simulink model "DCFastCharger"  (R2026b)
settings: Solver=ode23t  StopTime=simulation.simTime  MaxStep=1/(5*inverter.SwitchFrequency)  AbsTol=1e-3
PreLoadFcn:
  | run('DCFastChargerData.mlx');
undefined symbols (not defined in the file or in its folder): battery, inverter, rectifier
libraries: nesl_utility x34, fl_lib x22, ee_lib x14, eePwmGenerator x2, eeTransforms x2, batteryecm_lib x1, eeSinusoidalMeasurement x1, slpidlib x1, eePwmGeneratorThreeLevel x1, eePwmGeneratorTwoLevel x1, simulink_extras x1
(part 2 of 3)

== system DCFastCharger/EV Battery/EV Battery ==
  Battery (Table-Based) : batteryecm_lib/Battery (Table-Based)  PartSpecification="{\"CollectionId\":\"MW.SimscapeBatteryShared\",\"CollectionVersion\":\"1.0.0\",\"DatasetId\":\"Panasonic|NCR18650PF|simscape.battery.batteryTableBased\",\"DisplayName\":\"Panasonic:NCR18650PF\"}"  SOC_vec=[0 0.01 0.02 0.03 0.04 0.05 0.06 0.07 0.08 0.09 0.1 0.11 0.12 0.13 0.14 0.15 0.16 0.17 0.18 0.19 0.2 0.21 0.22 0.23 0.24 0.25 0.26 0.27 0.28 0.29 0.3 0.31 0.32 0.33 0.34 0.35 0.36 0.37 0.38 0.39 0.4 0.41 0.42 0.43 0.44 0.45 0.46 0.47 0.48 0.49 0.5 0.51 0.52 0.53 0.54 0.55 0.56 0.57 0.58 0.59 0.6 0.61 0.62 0.63 0.64 0.65 0.66 0.67 0.68 0.69 0.7 0.71 0.72 0.73 0.74 0.75 0.76 0.77 0.78 0.79 0.8 0.81 0.82 0.83 0.84 0.85 0.86 0.87 0.88 0.89 0.9 0.91 0.92 0.93 0.94 0.95 0.96 0.97 0.98 0.99 1]  T_dependence=simscape.enum.tablebattery.temperature_dependence.no  prm_dir=simscape.enum.tablebattery.prm_dir.noCurrentDirectionality  T_vec=[-10 0 25 45] degC  V0_mat=[2.9250925086225 2.9250925086225 2.9250925086225 2.9250925086225;3.02630036129653 3.02630036129653 3.02630036129653 3.02630036129653;3.10541208785785 3.10541208785785 3.10541208785785 3.10541208785785;3.16593241088406 3.16593241088406 3.16593241088406 3.16593241088406;3.21032916159511 3.21032916159511 3.21032916159511 3.21032916159511;3.25202417776279 3.25202417776279 3.25202417776279 3.25202417776279;3.27764615366987 3.27764615366987 3.27764615366987 3.27764615366987;3.30010470561178 3.30010470561178 3.30010470561178 3.30010470561178;3.32101021333279 3.32101021333279 3.32101021333279 3.32101021333279;3.33984622770258 3.33984622770258 3.33984622770258 3.33984622770258;3.35585830950675 3.35585830950675 3.35585830950675 3.35585830950675;3.37108925119603 3.37108925119603 3.37108925119603 3.37108925119603;3.3859421763038 3.3859421763038 3.3859421763038 3.3859421763038;3.39949357655528 3.39949357655528 3.39949357655528 3.39949357655528;3.41188533180246 3.41188533180246 3.41188533180246 3.41188533180246;3.42508750933082 3.42508750933082 3.42508750933082 3.42508750933082;3.43732483114827 3.43732483114827 3.43732483114827 3.43732483114827;3.44838610292672 3.44838610292672 3.44838610292672 3.44838610292672;3.45940404792364 3.45940404792364 3.45940404792364 3.45940404792364;3.46945718604369 3.46945718604369 3.46945718604369 3.46945718604369;3.4756511424782 3.4756511424782 3.4756511424782 3.4756511424782;3.48092723774567 3.48092723774567 3.48092723774567 3.48092723774567;3.48828844475697 3.48828844475697 3.48828844475697 3.48828844475697;3.49727445600775 3.49727445600775 3.49727445600775 3.49727445600775;3.50602219248741 3.50602219248741 3.50602219248741 3.50602219248741;3.51277142257531 3.51277142257531 3.51277142257531 3.51277142257531;3.5189897231308 3.5189897231308 3.5189897231308 3.5189897231308;3.52519494567954 3.52519494567954 3.52519494567954 3.52519494567954;3.53104467138329 3.53104467138329 3.53104467138329 3.53104467138329;3.53631377637871 3.53631377637871 3.53631377637871 3.53631377637871;3.54093819602626 3.54093819602626 3.54093819602626 3.54093819602626;3.54463024006975 3.54463024006975 3.54463024006975 3.54463024006975;3.54855792050501 3.54855792050501 3.54855792050501 3.54855792050501;3.55281403232742 3.55281403232742 3.55281403232742 3.55281403232742;3.55817391786706 3.55817391786706 3.55817391786706 3.55817391786706;3.56415253483575 3.56415253483575 3.56415253483575 3.56415253483575;3.56997687090312 3.56997687090312 3.56997687090312 3.56997687090312;3.57540644773372 3.57540644773372 3.57540644773372 3.57540644773372;3.58072477562415 3.58072477562415 3.58072477562415 3.58072477562415;3.58617648767287 3.58617648767287 3.58617648767287 3.58617648767287;3.59255537492352 3.59255537492352 3.59255537492352 3.59255537492352;3.59925786836004 3.59925786836004 3.59925786836004 3.59925786836004;3.6059599902444 3.6059599902444 3.6059599902444 3.6059599902444;3.61253369195548 3.61253369195548 3.61253369195548 3.61253369195548;3.61908508495676 3.61908508495676 3.61908508495676 3.61908508495676;3.62459685737123 3.62459685737123 3.62459685737123 3.62459685737123;3.62997084407271 3.62997084407271 3.62997084407271 3.62997084407271;3.63600645659379 3.63600645659379 3.63600645659379 3.63600645659379;3.64260961230588 3.64260961230588 3.64260961230588 3.64260961230588;3.64905571343015 3.64905571343015 3.64905571343015 3.64905571343015;3.65538413005486 3.65538413005486 3.65538413005486 3.65538413005486;3.66209665206491 3.66209665206491 3.66209665206491 3.66209665206491;3.66960310665593 3.66960310665593 3.66960310665593 3.66960310665593;3.67782215533979 3.67782215533979 3.67782215533979 3.67782215533979;3.68577251249088 3.68577251249088 3.68577251249088 3.68577251249088;3.69607105582974 3.69607105582974 3.69607105582974 3.69607105582974;3.70665559836365 3.70665559836365 3.70665559836365 3.70665559836365;3.71697762414446 3.71697762414446 3.71697762414446 3.71697762414446;3.72601099321076 3.72601099321076 3.72601099321076 3.72601099321076 ...(+2844 chars)] V  V0_vec=[2.9250925086225 3.02630036129653 3.10541208785785 3.16593241088406 3.21032916159511 3.25202417776279 3.27764615366987 3.30010470561178 3.32101021333279 3.33984622770258 3.35585830950675 3.37108925119603 3.3859421763038 3.39949357655528 3.41188533180246 3.42508750933082 3.43732483114827 3.44838610292672 3.45940404792364 3.46945718604369 3.4756511424782 3.48092723774567 3.48828844475697 3.49727445600775 3.50602219248741 3.51277142257531 3.5189897231308 3.52519494567954 3.53104467138329 3.53631377637871 3.54093819602626 3.54463024006975 3.54855792050501 3.55281403232742 3.55817391786706 3.56415253483575 3.56997687090312 3.57540644773372 3.58072477562415 3.58617648767287 3.59255537492352 3.59925786836004 3.6059599902444 3.61253369195548 3.61908508495676 3.62459685737123 3.62997084407271 3.63600645659379 3.64260961230588 3.64905571343015 3.65538413005486 3.66209665206491 3.66960310665593 3.67782215533979 3.68577251249088 3.69607105582974 3.70665559836365 3.71697762414446 3.72601099321076 3.73441114732962 3.74311002352401 3.75294627542582 3.76247271262466 3.77151242602685 3.78040087631196 3.79005401630221 3.79990949046456 3.80976496462691 3.81844612732862 3.82578802176443 3.83313829687425 3.84080281949238 3.84973459076441 3.85949329030869 3.86965559240319 3.87924489617679 3.88819434423151 3.89590288247261 3.90359081518304 3.91379255081804 3.92466354434184 3.9366161325385 3.95005027786179 3.96305146054116 3.97214053014382 3.98120257186703 3.99267995044399 4.0057555337863 4.0188391070389 4.03188069898376 4.04441045486762 4.05587613526738 4.06606826108443 4.07458148513164 4.08216556084643 4.08994198301214 4.10139357870482 4.11503704946696 4.13270033629767 4.15282395048316 4.17387289866414] V  V_range=[0, inf] V  R0_mat=[0.158948722548683 0.155965220476233 0.0642584048974491 0.156271637839508;0.164094056100913 0.155561872039019 0.0643716270460056 0.0958858667534425;0.16590247791362 0.150196791550074 0.063971690534484 0.0735783105788718;0.164336402457897 0.145157421371546 0.0634227939708557 0.0603478425562904;0.162194103534027 0.137561513429308 0.0626187357617236 0.0554701940184629;0.161368428396527 0.132847642820159 0.0622925177341011 0.0565695495484196;0.154034534555668 0.126124135972156 0.0608902569786277 0.0547834384667639;0.150348957772332 0.11992991718736 0.0592086978048456 0.0546076326919676;0.146678161591533 0.114221598629678 0.0583937154824633 0.0553174331388643;0.143764862122133 0.1117675900648 0.057496531429448 0.0567839252512895;0.141557404155717 0.108267680549691 0.0573966942403751 0.0568973079738719;0.139111638730854 0.10588448132351 0.0571494121217046 0.0563386051707534;0.137029789271551 0.10371863599948 0.0568904518955565 0.0568492069290691;0.134465893569179 0.102157603100912 0.0566162508651665 0.0573623269867748;0.133579806251124 0.101182159975048 0.0563201629222844 0.0575820103565126;0.133163032374253 0.100506873249622 0.0564506791916006 0.0591218449352567;0.132701252660884 0.099863696339387 0.0563243957272469 0.0603043255469938;0.131974699165714 0.0988544564628729 0.0561368224553059 0.0604335920006752;0.131283115762638 0.098955481127068 0.0562749855286881 0.0603849408722603;0.130548646804137 0.099375021703539 0.0562019955818807 0.0601584729212836;0.128384851295437 0.0983652357298114 0.0555274629478928 0.0592378223566733;0.126118815339946 0.0970669163577878 0.0546888535605859 0.0579772232116761;0.125402797723443 0.0966018361754667 0.054265365781618 0.057400894490884;0.125288559454898 0.096738535341105 0.0540037545839983 0.0569904797117699;0.125047401593192 0.0967965349271084 0.0536899957091979 0.0564918150174259;0.124051599285487 0.0961581839164014 0.0533086284567699 0.0554970632508009;0.12285915641022 0.0953231923381314 0.0530642654231626 0.054870770374079;0.122165505140544 0.094483357053662 0.0528170401995282 0.0542396337911578;0.121494072509647 0.0935118562710458 0.0525235778530978 0.053212217478928;0.120601470615727 0.0925622611521829 0.0520471214590463 0.0519633792021407;0.119286253401761 0.091460027942767 0.0514017212712578 0.0507774032613698;0.117625711889992 0.0900124704355474 0.0505504728406427 0.0494999445481573;0.116099177219541 0.088652185666025 0.049830956429225 0.0490253291641116;0.114900842886945 0.0876321360266284 0.0493618778947113 0.0489723769096966;0.114111313634808 0.0873497188498393 0.0490976398787349 0.0493282297357397;0.113550944171205 0.0872964614615855 0.048915118220372 0.0492640332618821;0.112988973186793 0.0871860629987678 0.048614953173201 0.0489039680872592;0.112297629639516 0.0869949880800038 0.0482896295727264 0.048407984264869;0.111565082781067 0.0870678281013333 0.0479473144926267 0.048233027492356;0.110761242109476 0.0871900696627706 0.0477067084656926 0.0481074722599508;0.110212729124657 0.0876557094471428 0.0476555994749632 0.0483253152504805;0.109784070282755 0.0873084934166727 0.0476617367023012 0.0482979562377831;0.109503678016475 0.0860654941887924 0.0476677926135098 0.0477344062008158;0.109268014836562 0.0847749319337712 0.0476696468980676 0.0471232931367077;0.109024089171536 0.0838029485664093 0.0476752475967437 0.0465039175874869;0.108621493141403 0.0835326079948486 0.0474506512594163 0.0461687494231811;0.108259397918414 0.0832112356777327 0.0471837257520344 0.0458650723508987;0.108008944918365 0.0831349099604705 0.0468394367793266 0.0455774893634449;0.107209504544399 0.082814101209584 0.0466240014760817 0.0450730540518787;0.106351895804571 0.0823498486862532 0.0464022435243735 0.0445104503744493;0.105450700213058 0.0818420093112374 0.0461547297057605 0.043898896196232;0.104474728336867 0.0815181360390074 0.045579722159839 0.0433287006666967;0.103783729089634 0.0816852711857715 0.0450589645831341 0.0430525542412283;0.103537470985121 0.0821163300706208 0.044701216779163 ...(+3502 chars)] Ohm  R0_vec=[0.0642584048974491 0.0643716270460056 0.063971690534484 0.0634227939708557 0.0626187357617236 0.0622925177341011 0.0608902569786277 0.0592086978048456 0.0583937154824633 0.057496531429448 0.0573966942403751 0.0571494121217046 0.0568904518955565 0.0566162508651665 0.0563201629222844 0.0564506791916006 0.0563243957272469 0.0561368224553059 0.0562749855286881 0.0562019955818807 0.0555274629478928 0.0546888535605859 0.054265365781618 0.0540037545839983 0.0536899957091979 0.0533086284567699 0.0530642654231626 0.0528170401995282 0.0525235778530978 0.0520471214590463 0.0514017212712578 0.0505504728406427 0.049830956429225 0.0493618778947113 0.0490976398787349 0.048915118220372 0.048614953173201 0.0482896295727264 0.0479473144926267 0.0477067084656926 0.0476555994749632 0.0476617367023012 0.0476677926135098 0.0476696468980676 0.0476752475967437 0.0474506512594163 0.0471837257520344 0.0468394367793266 0.0466240014760817 0.0464022435243735 0.0461547297057605 0.045579722159839 0.0450589645831341 0.044701216779163 0.0443326520857887 0.0445314146147127 0.045015739502721 0.0454894960834381 0.0456812234168713 0.0456928203147297 0.0455424443466032 0.0455233887186122 0.0454918606790689 0.0454039925420258 0.0452830196823913 0.0453842814819192 0.0455361622547251 0.0456880430275314 0.0456524416563551 0.0454382214701634 0.0452225970388179 0.0450757473146783 0.0448448857727635 0.0447127937510717 0.0447342410972344 0.0448403278985325 0.0450878835664416 0.0450853981911946 0.0450820832857262 0.0456224791026564 0.0458434697709894 0.046286077419994 0.0470885819136486 0.0477828468023542 0.0475520781260466 0.0472569254085986 0.0474663234338054 0.0479591925321213 0.0484565832495922 0.0490028384423885 0.0495284883187202 0.0497251543915884 0.0496855026515378 0.0492826811538264 0.0486578614415746 0.0474486947337877 0.0465126146130306 0.0457818101518658 0.0456572937139443 0.0412205205929347 0.0351051518441569] Ohm  R0_dis_mat=[0.03 0.015 0.002;0.04 0.017 0.008;0.039 0.012 0.006;0.027 0.013 0.021] % Parameter not set Ohm  R0_dis_vec=[0.015 0.017 0.012 0.013] % Parameter not set Ohm  R0_ch_mat=[0.03 0.015 0.002;0.04 0.017 0.008;0.039 0.012 0.006;0.027 0.013 0.021] % Parameter not set Ohm  R0_ch_vec=[0.015 0.017 0.012 0.013] % Parameter not set Ohm  AH=2.73516665928367 hr*A  prm_leak=simscape.enum.tablebattery.prm_leak.disabled  Rleak_vec=[8000 7000 6000] % Parameter not set Ohm  Rleak=7000 % Parameter not set Ohm  extrapolation_option=simscape.enum.extrapolation.nearest  SOC_port=simscape.enum.tablebattery.enable.yes  prm_dyn=simscape.enum.tablebattery.prm_dyn.off  R1_mat=[0.089 0.076 0.01;0.042 0.022 0.099;0.019 0.007 0.002;0.051 0.043 0.029] % Parameter not set Ohm  R1_vec=[0.076 0.022 0.007 0.043] % Parameter not set Ohm  tau1_mat=[44 148 235;93 110 1000;19 27 133;0.5 22 3] % Parameter not set s  tau1_vec=[148 110 27 22] % Parameter not set s  R2_mat=[0.014 0.382 0.407;0.028 0.006 0.007;0.014 0.007 0.006;0.333 0.956 0.912] % Parameter not set Ohm  R2_vec=[0.382 0.006 0.007 0.956] % Parameter not set Ohm  tau2_mat=[1 44 5644;11 24 506;2 14 330;3310 13419 30216] % Parameter not set s  tau2_vec=[44 24 14 13419] % Parameter not set s  R3_mat=[0.014 0.382 0.407;0.028 0.006 0.007;0.014 0.007 0.006;0.333 0.956 0.912] % Parameter not set Ohm  R3_vec=[0.382 0.006 0.007 0.956] % Parameter not set Ohm  tau3_mat=[1 44 5644;11 24 506;2 14 330;3310 13419 30216] % Parameter not set s  tau3_vec=[44 24 14 13419] % Parameter not set s  R4_mat=[0.014 0.382 0.407;0.028 0.006 0.007;0.014 0.007 0.006;0.333 0.956 0.912] % Parameter not set Ohm  R4_vec=[0.382 0.006 0.007 0.956] % Parameter not set Ohm  tau4_mat=[1 44 5644;11 24 506;2 14 330;3310 13419 30216] % Parameter not set s  tau4_vec=[44 24 14 13419] % Parameter not set s  R5_mat=[0.014 0.382 0.407;0.028 0.006 0.007;0.014 0.007 0.006;0.333 0.956 0.912] % Parameter not set Ohm  R5_vec=[0.382 0.006 0.007 0.956] % Parameter not set Ohm  tau5_mat=[1 44 5644;11 24 506;2 14 330;3310 13419 30216] % Parameter not set s  tau5_vec=[44 24 14 13419] % Parameter not set s  prm_fade=simscape.enum.tablebattery.prm_fade.tableN  N0=100 % Parameter not set  dV0=0 % Parameter not set  dR0=0 % Parameter not set  dAH=0 % Parameter not set  dRleak=0 % Parameter not set  dR1=0 % Parameter not set  dR2=0 % Parameter not set  dR3=0 % Parameter not set  dR4=0 % Parameter not set  dR5=0 % Parameter not set  N0vec=[1 7 13 19 25 31 37 43 49 55 61 67 73 79 85 91 97 103 109 115 121 127 133 139 145 151 157 163 169 175 181 187 193 199 205 211 217 223 229 235 241 247 253 259 265 271 277 283 289 295 301 307 313 319 325 331 337 343 349 355 361 367 373 379 385 391 397 403 409 415 421 427 433 439 445 451 457 463 469 475 481 487 493 499]  Tfadevec=[298.15 323.15] % Parameter not set K  dV0vec=[0 -0.205322446679001 -0.410644893358002 -0.611058438675835 -0.807354693721955 -1.0015461710045 -1.17384310657063 -1.34614004213677 -1.47740012287432 -1.58387836723114 -1.690356611588 -1.78714189934731 -1.87651401189101 -1.96588612443468 -2.04101080690197 -2.10170062652461 -2.16239044614726 -2.21633350400211 -2.26428234838279 -2.31223119276347 -2.36018003714415 -2.41171229286392 -2.46553549695213 -2.51935870104035 -2.57318190512856 -2.64508715419502 -2.72179418719877 -2.79850122020252 -2.88122798263413 -2.96751992414094 -3.05381186564772 -3.14366470722484 -3.23796499505138 -3.33226528287793 -3.38092510003549 -3.4273752475407 -3.47468340383756 -3.52199156013442 -3.56929971643126 -3.61660787272814 -3.663916029025 -3.71122418532186 -3.76958571632676 -3.83114472817411 -3.89270374002147 -3.95426275186883 -4.01582176371619 -4.07735052835229 -4.13887194718341 -4.20039336601454 -4.26007865261728 -4.31160679119979 -4.36044442770985 -4.40567437565134 -4.45090432359283 -4.49613427153431 -4.54136421947579 -4.58659416741728 -4.62903918136233 -4.6691583474524 -4.70927751354245 -4.74939667963251 -4.78951584572256 -4.82963501181263 -4.86986314897544 -4.91010197198366 -4.95034079499188 -4.98044487353192 -4.99960776219833 -5.01877065086475 -5.03793353953117 -5.05972954523592 -5.08714051545705 -5.11455148567819 -5.14196245589932 -5.17147950123752 -5.20235900192375 -5.23323850260996 -5.26411800329619 -5.29499750398241 -5.32587700466864 -5.35675650535486 -5.38847412791779 -5.42038197122406]  dR0vec=[0;0;0;0;0;0;0;0;0;0;0;0;0;0;0;0;0;0;0;0;0;0;0;0;0;0;0;0;0;0;0;0;0;0;0;0;0;0;0;0;0;0;0;0;0;0;0;0;0;0;0;0;0;0;0;0;0;0;0;0;0;0;0;0;0;0;0;0;0;0;0;0;0;0;0;0;0;0;0;0;0;0;0;0] % Parameter not set  dAHvec=[0 -0.407141386976734 -0.814282773953468 -1.22142416093019 -1.62856554790692 -2.03570693488365 -2.44284832186039 -2.84998970883712 -3.20734856882233 -3.53309167786423 -3.85883478690612 -4.18457789594802 -4.51032100498989 -4.8360641140318 -5.1618072230737 -5.48755033211559 -5.81329344115748 -6.10543218183984 -6.36931718194932 -6.63320218205879 -6.89708718216827 -7.16097218227776 -7.42485718238722 -7.6887421824967 -7.95262718260619 -8.25489660762765 -8.56902676255148 -8.8831569174753 -9.19728707239912 -9.51141722732295 -9.82554738224679 -10.1396775371706 -10.4538076920944 -10.7679378470183 -10.9300319005421 -11.0814384407007 -11.2328449808593 -11.3842515210179 -11.5356580611765 -11.6870646013351 -11.8384711414938 -11.9898776816524 -12.176092947695 -12.3724762187309 -12.5688594897668 -12.7652427608027 -12.9616260318386 -13.1580093028745 -13.3543925739104 -13.5507758449463 -13.7412979759122 -13.9057815752421 -14.0702651745719 -14.2347487739018 -14.3992323732316 -14.5637159725615 -14.7281995718913 -14.8926831712212 -15.0595765368119 -15.2443608328623 -15.4291451289128 -15.6139294249632 -15.7987137210137 -15.9834980170641 -16.1682823131146 -16.353066609165 -16.5378509052155 -16.6760945352573 -16.7640941492568 -16.8520937632563 -16.9400933772558 -17.0280929912553 -17.1160926052547 -17.2040922192542 -17.2920918332537 -17.3868527474137 -17.4859876601498 -17.585122572886 -17.6842574856221 -17.7833923983582 -17.8825273110943 -17.9816622238304 -18.0807971365665 -18.1799320493027]  dRleakvec=[0 0 0] % Parameter not set  dR1vec=[0 0 0] % Parameter not set  dR2vec=[0 0 0] % Parameter not set  dR3vec=[0 0 0] % Parameter not set  dR4vec=[0 0 0] % Parameter not set  dR5vec=[0 0 0] % Parameter not set  dV0mat=[0 0;0 0;0 0] % Parameter not set  dR0mat=[0 0;0 0;0 0] % Parameter not set  dAHmat=[0 0;0 0;0 0] % Parameter not set  dRleakmat=[0 0;0 0;0 0] % Parameter not set  dR1mat=[0 0;0 0;0 0] % Parameter not set  dR2mat=[0 0;0 0;0 0] % Parameter not set  dR3mat=[0 0;0 0;0 0] % Parameter not set  dR4mat=[0 0;0 0;0 0] % Parameter not set  dR5mat=[0 0;0 0;0 0] % Parameter not set  prm_age_modeling=simscape.enum.tablebattery.prm_age_modeling.equation  storage_dt_age_vec=0 % Parameter not set d  storage_T_age_vec=273 % Parameter not set K  prm_age_OCV=simscape.enum.tablebattery.prm_age_OCV.SOC  OCV_age=0.9 % Parameter not set  SOC_age=0.6 % Parameter not set  prm_age_resistance=simscape.enum.tablebattery.prm_age.disabled  OCV_scaling_age_resistance=2213400  OCV_offset_age_resistance=1632000  temp_exp_age_resistance=0.515833569 V  t_exp_age_resistance=0.75  T_age_vec_resistance=[273.15 298.15 323.15] K  dt_age_vec_resistance=[90 180 270 360] d  dR0_age_vec=[0 0 0] % Parameter not set  t_meas_dR0_age=100 % Parameter not set d  dR0_age_mat=[0 0 0;0 0 0;0 0 0;0 0 0] % Parameter not set  prm_age_capacity=simscape.enum.tablebattery.prm_age.disabled  OCV_scaling_age_capacity=1.5097e07  OCV_offset_age_capacity=8.3625e06  temp_exp_age_capacity=0.6011 V  t_exp_age_capacity=0.75  T_age_vec_capacity=[273.15, 298.15, 323.15] K  dt_age_vec_capacity=[90, 180, 270, 360] d  dAH_age_vec=[0, 0, 0]  t_meas_dAH_age=100 d  dAH_age_mat=[0, 0, 0; 0, 0, 0; 0, 0, 0; 0, 0, 0]  thermal_port=simscape.enum.thermaleffects.omit  temperature=298.15 K  thermal_mass=30000 J/K  i_specify=off  i_priority=None  i=0 A  i_nominal_specify=off  i_nominal_value=1  i_nominal_unit=A  v_specify=off  v_priority=None  v=0 V  v_nominal_specify=off  v_nominal_value=1  v_nominal_unit=V  stateOfCharge_specify=on  stateOfCharge_priority=High  stateOfCharge=battery.initialSOC  stateOfCharge_nominal_specify=off  stateOfCharge_nominal_value=1  stateOfCharge_nominal_unit=1  num_cycles_specify=off  num_cycles_priority=High  num_cycles=0  num_cycles_nominal_specify=off  num_cycles_nominal_value=1  num_cycles_nominal_unit=1  cell_temperature_specify=off  cell_temperature_priority=High  cell_temperature=298.15 K  cell_temperature_nominal_specify=off  cell_temperature_nominal_value=1  cell_temperature_nominal_unit=K
      settings: AttributesFormatString=Panasonic:NCR18650PF
  "Number of cells in series " : fl_lib/Electrical/Electrical Sources/Voltage-Controlled Voltage Source  K=-1*battery.cellsInSeries  v1_specify=off  v1_priority=None  v1=0 V  v1_nominal_specify=off  v1_nominal_value=1  v1_nominal_unit=V  v2_specify=off  v2_priority=None  v2=0 V  v2_nominal_specify=off  v2_nominal_value=1  v2_nominal_unit=V
  Number of strings in parallel : fl_lib/Electrical/Electrical Sources/Current-Controlled Current Source  K=-1*(battery.batteryStringsInParallel-1)  i1_specify=off  i1_priority=None  i1=0 A  i1_nominal_specify=off  i1_nominal_value=1  i1_nominal_unit=A  i2_specify=off  i2_priority=None  i2=0 A  i2_nominal_specify=off  i2_nominal_value=1  i2_nominal_unit=A
  PS-Simulink Converter : nesl_utility/PS-Simulink Converter  PhysicalDomain=network_engine_domain  SubClassName=ps_output  LeftPortType=input  RightPortType=output  PseudoPeriodic=off  Frequencies=[]  VectorFormat=1-D array  Unit=inherit  AffineConversion=off
  + : PMIOPort  Side=Left
  - : PMIOPort  Port=2  Side=Right
  SOC : Outport
  wires:
  PS-Simulink Converter/1 -> SOC/1
  connections:
  "Number of cells in series "/RConn2 -- "Number of cells in series "/RConn1 -- Battery (Table-Based)/LConn1
  "Number of cells in series "/LConn1 -- Number of strings in parallel/LConn2 -- -/RConn1 -- Battery (Table-Based)/RConn1
  Number of strings in parallel/RConn1 -- Number of strings in parallel/RConn2 -- +/RConn1
  Number of strings in parallel/LConn1 -- "Number of cells in series "/LConn2
  PS-Simulink Converter/LConn1 -- Battery (Table-Based)/LConn2

== system DCFastCharger/EV Battery/i ==
  Current Sensor : fl_lib/Electrical/Electrical Sensors/Current Sensor
  PS-Simulink Converter1 : nesl_utility/PS-Simulink Converter  PhysicalDomain=network_engine_domain  SubClassName=ps_output  LeftPortType=input  RightPortType=output  PseudoPeriodic=off  Frequencies=[]  VectorFormat=1-D array  Unit=1  AffineConversion=off
  Rate Transition : RateTransition  OutPortSampleTime=1/(10*inverter.SwitchFrequency)
  + : PMIOPort  Side=Left
  - : PMIOPort  Port=2  Side=Right
  I : Outport
  wires:
  Rate Transition/1 -> I/1
  PS-Simulink Converter1/1 -> Rate Transition/1
  connections:
  Current Sensor/RConn1 -- PS-Simulink Converter1/LConn1
  Current Sensor/RConn2 -- -/RConn1
  Current Sensor/LConn1 -- +/RConn1

== system DCFastCharger/EV Battery/v ==
  PS-Simulink Converter : nesl_utility/PS-Simulink Converter  PhysicalDomain=network_engine_domain  SubClassName=ps_output  LeftPortType=input  RightPortType=output  PseudoPeriodic=off  Frequencies=[]  VectorFormat=1-D array  Unit=1  AffineConversion=off
  Rate Transition : RateTransition  OutPortSampleTime=1/(10*inverter.SwitchFrequency)
  Voltage Sensor : fl_lib/Electrical/Electrical Sensors/Voltage Sensor
  + : PMIOPort  Side=Right
  - : PMIOPort  Port=2  Side=Left
  V : Outport
  wires:
  PS-Simulink Converter/1 -> Rate Transition/1
  Rate Transition/1 -> V/1
  connections:
  +/RConn1 -- Voltage Sensor/LConn1
  -/RConn1 -- Voltage Sensor/RConn2
  Voltage Sensor/RConn1 -- PS-Simulink Converter/LConn1

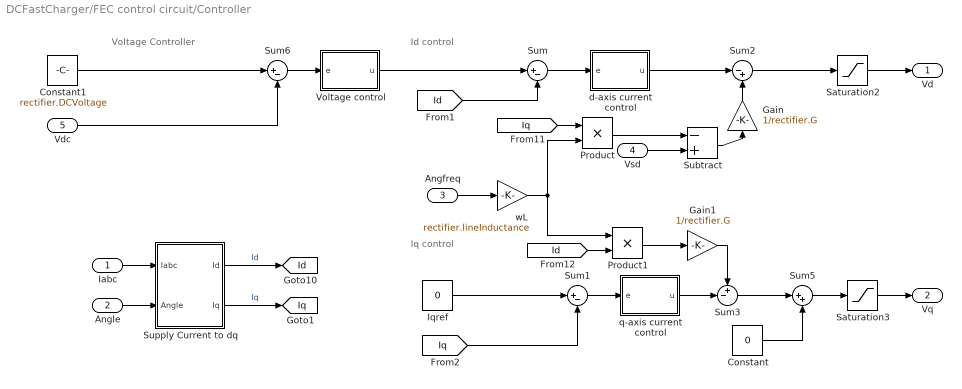
== system DCFastCharger/FEC control circuit/Controller ==
  note: Id control
  note: Voltage Controller
  note: Iq control
  Iabc : Inport
  Angle : Inport  Port=2
  Angfreq : Inport  Port=3
  Vsd : Inport  Port=4
  Vdc : Inport  Port=5
  Constant : Constant  Value=0
  Constant1 : Constant  Value=rectifier.DCVoltage
  Gain : Gain  Gain=1/rectifier.G
  Gain1 : Gain  Gain=1/rectifier.G
  Iqref : Constant  Value=0
  Product : Product
  Product1 : Product
  Saturation2 : Saturate  UpperLimit=4  LowerLimit=-3
  Saturation3 : Saturate  UpperLimit=1  LowerLimit=-1
  Subtract : Sum  Inputs=-+
  Sum : Sum  Inputs=|+-
  Sum1 : Sum  Inputs=|+-
  Sum2 : Sum  Inputs=|-+
  Sum3 : Sum  Inputs=+-|
  Sum5 : Sum  Inputs=|++
  Sum6 : Sum  Inputs=|+-
  Supply Current to dq : Subsystem
  Voltage control : Subsystem
  d-axis current control : Subsystem
  q-axis current control : Subsystem
  wL : Gain  Gain=rectifier.lineInductance
  Vd : Outport  VectorParamsAs1DForOutWhenUnconnected=off
  Vq : Outport  Port=2  VectorParamsAs1DForOutWhenUnconnected=off
  tag scope: Id=global, Iq=global
  wires:
  Sum1/1 -> q-axis current control/1(e)
  wL/1 -> Product/2, Product1/1
  [Id] -> Product1/2
  [Iq] -> Product/1
  Sum3/1 -> Sum5/1
  Sum2/1 -> Saturation2/1
  Sum5/1 -> Saturation3/1
  Angfreq/1 -> wL/1
  Constant/1 -> Sum5/2
  Vdc/1 -> Sum6/2
  Sum/1 -> d-axis current control/1(e)
  [Id] -> Sum/2
  d-axis current control/1(u) -> Sum2/1
  q-axis current control/1(u) -> Sum3/2
  Supply Current to dq/1(Id) -> [Id]  "Id"
  Supply Current to dq/2(Iq) -> [Iq]  "Iq"
  Sum6/1 -> Voltage control/1(e)
  Saturation3/1 -> Vq/1
  Saturation2/1 -> Vd/1
  Iqref/1 -> Sum1/1
  [Iq] -> Sum1/2
  Voltage control/1(u) -> Sum/1
  Constant1/1 -> Sum6/1
  Product1/1 -> Gain1/1
  Product/1 -> Subtract/1
  Vsd/1 -> Subtract/2
  Subtract/1 -> Gain/1
  Gain/1 -> Sum2/2
  Gain1/1 -> Sum3/1
  Iabc/1 -> Supply Current to dq/1(Iabc)
  Angle/1 -> Supply Current to dq/2(Angle)

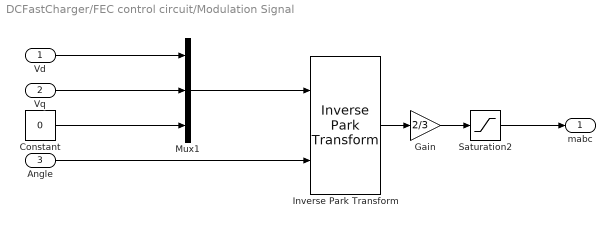
== system DCFastCharger/FEC control circuit/Modulation Signal ==
  Vd : Inport
  Vq : Inport  Port=2
  Angle : Inport  Port=3
  Constant : Constant  Value=0
  Gain : Gain  Gain=2/3
  Inverse Park Transform : eeTransforms/Inverse Park Transform  AxisAlignment=D-axis  PowerInvariant=off
  Mux1 : Mux  Inputs=3
  Saturation2 : Saturate  UpperLimit=1  LowerLimit=-1
  mabc : Outport  VectorParamsAs1DForOutWhenUnconnected=off
  wires:
  Gain/1 -> Saturation2/1
  Mux1/1 -> Inverse Park Transform/1
  Inverse Park Transform/1 -> Gain/1
  Constant/1 -> Mux1/3
  Vd/1 -> Mux1/1
  Vq/1 -> Mux1/2
  Angle/1 -> Inverse Park Transform/2
  Saturation2/1 -> mabc/1

== system DCFastCharger/Filter & AC measurements/PLL ==
  Vabc : Inport
  Constant : Constant  Value=pi/2
  Gain2 : Gain  Gain=2*pi
  "Sinusoidal measurement (PLL, Three-Phase)" : eeSinusoidalMeasurement/Sinusoidal Measurement (PLL, Three-Phase)  Kp_LF=0.05  Ki_LF=1  F0=rectifier.SystemFrequency  Theta0=0  Ts=rectifier.VoltageSensorT
  Subtract : Sum  Inputs=-+
  Vphm to Vsd : Gain  Gain=3/2
  w : Outport  VectorParamsAs1DForOutWhenUnconnected=off
  angle : Outport  Port=2  VectorParamsAs1DForOutWhenUnconnected=off
  Vsd : Outport  Port=3  VectorParamsAs1DForOutWhenUnconnected=off
  wires:
  "Sinusoidal measurement (PLL, Three-Phase)"/3 -> Vphm to Vsd/1
  Gain2/1 -> w/1
  "Sinusoidal measurement (PLL, Three-Phase)"/1 -> Gain2/1
  Vabc/1 -> "Sinusoidal measurement (PLL, Three-Phase)"/1
  Subtract/1 -> angle/1
  "Sinusoidal measurement (PLL, Three-Phase)"/2 -> Subtract/2
  Constant/1 -> Subtract/1
  Vphm to Vsd/1 -> Vsd/1

== system DCFastCharger/Front end converter/DC bus current sensor ==
  Current Sensor : fl_lib/Electrical/Electrical Sensors/Current Sensor
      settings: LogSimulationData=on
  PS-Simulink Converter1 : nesl_utility/PS-Simulink Converter  PhysicalDomain=network_engine_domain  SubClassName=ps_output  LeftPortType=input  RightPortType=output  PseudoPeriodic=off  Frequencies=[]  VectorFormat=1-D array  Unit=1  AffineConversion=off
  Sensor dynamics : TransferFcn  Numerator=1  Denominator=[1/(10*rectifier.SwitchFrequency) 1]
  + : PMIOPort  Side=Left
  - : PMIOPort  Port=2  Side=Right
  I : Outport
  wires:
  PS-Simulink Converter1/1 -> Sensor dynamics/1
  Sensor dynamics/1 -> I/1
  connections:
  Current Sensor/LConn1 -- +/RConn1
  PS-Simulink Converter1/LConn1 -- Current Sensor/RConn1
  Current Sensor/RConn2 -- -/RConn1

== system DCFastCharger/Front end converter/FEC ==
  m : Inport
  Vdc : Inport  Port=2
  Average : Subsystem  VariantControl=powerCircuit==0
  Three Level : Subsystem  VariantControl=powerCircuit==2
  Two Level : Subsystem  VariantControl=powerCircuit==1
  + : PMIOPort  Side=Right
  O : PMIOPort  Port=2  Side=Right
  - : PMIOPort  Port=3  Side=Right
  ABC : PMIOPort  Port=4  Side=Left

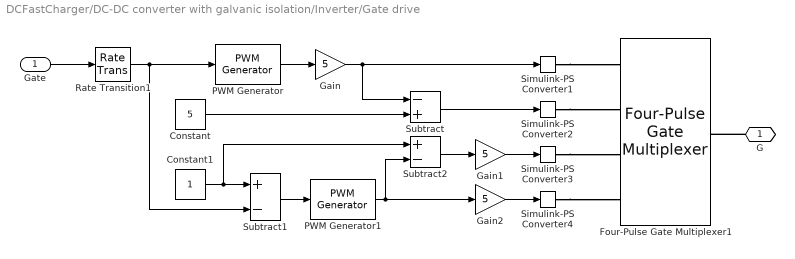
== system DCFastCharger/DC-DC converter with galvanic isolation/Inverter/Gate drive ==
  Gate : Inport
  Constant : Constant  Value=5
  Constant1 : Constant
  Four-Pulse Gate Multiplexer1 : ee_lib/Semiconductors & Converters/Converters/Four-Pulse Gate Multiplexer  port_option=ee.enum.controlport.ps
  Gain : Gain  Gain=5
  Gain1 : Gain  Gain=5
  Gain2 : Gain  Gain=5
  PWM Generator : eePwmGenerator/PWM Generator  CarrCount=Up  Tper=1/inverter.SwitchFrequency  Tdelay=0  Ts=1/(10*inverter.SwitchFrequency)
  PWM Generator1 : eePwmGenerator/PWM Generator  CarrCount=Up  Tper=1/inverter.SwitchFrequency  Tdelay=0  Ts=1/(10*inverter.SwitchFrequency)
  Rate Transition1 : RateTransition  OutPortSampleTime=1/(10*inverter.SwitchFrequency)
  Simulink-PS Converter{1..4} (4 alike) : nesl_utility/Simulink-PS Converter  PhysicalDomain=network_engine_domain  SubClassName=ps_input  LeftPortType=input  RightPortType=output  PseudoPeriodic=off  Frequencies=[]  NoiseDistribution=none  NoiseParameters=[]  Unit=1  AffineConversion=off  FilteringAndDerivatives=provide  SimscapeFilterOrder=1  InputFilterTimeConstant=0.001  UdotUserProvided=0
  Subtract : Sum  Inputs=-+
  Subtract1 : Sum  Inputs=+-
  Subtract2 : Sum  Inputs=+-
  G : PMIOPort  Side=Right
  wires:
  Rate Transition1/1 -> PWM Generator/1, Subtract1/2
  PWM Generator/1 -> Gain/1
  Constant/1 -> Subtract/2
  Gain/1 -> Simulink-PS Converter1/1, Subtract/1
  Subtract1/1 -> PWM Generator1/1
  PWM Generator1/1 -> Subtract2/2, Gain2/1
  Subtract/1 -> Simulink-PS Converter2/1
  Gain2/1 -> Simulink-PS Converter4/1
  Gate/1 -> Rate Transition1/1
  Subtract2/1 -> Gain1/1
  Gain1/1 -> Simulink-PS Converter3/1
  Constant1/1 -> Subtract2/1, Subtract1/1
  connections:
  G/RConn1 -- Four-Pulse Gate Multiplexer1/RConn1
  Simulink-PS Converter1/RConn1 -- Four-Pulse Gate Multiplexer1/LConn1
  Simulink-PS Converter2/RConn1 -- Four-Pulse Gate Multiplexer1/LConn2
  Simulink-PS Converter4/RConn1 -- Four-Pulse Gate Multiplexer1/LConn4
  Simulink-PS Converter3/RConn1 -- Four-Pulse Gate Multiplexer1/LConn3

== system DCFastCharger/FEC control circuit/Controller/Supply Current to dq ==
  Iabc : Inport
  Angle : Inport  Port=2
  Demux : Demux  Outputs=3
  Gain1 : Gain  Gain=1.5
  Park Transform : eeTransforms/Park Transform  AxisAlignment=D-axis  PowerInvariant=off
  Terminator : Terminator
  Id : Outport  VectorParamsAs1DForOutWhenUnconnected=off
  Iq : Outport  Port=2  VectorParamsAs1DForOutWhenUnconnected=off
  wires:
  Demux/3 -> Terminator/1
  Gain1/1 -> Demux/1
  Park Transform/1 -> Gain1/1
  Demux/2 -> Iq/1
  Demux/1 -> Id/1
  Iabc/1 -> Park Transform/1
  Angle/1 -> Park Transform/2

== system DCFastCharger/FEC control circuit/Controller/Voltage control ==
  e : Inport
  Integrator : Integrator  LimitOutput=on  UpperSaturationLimit=500  LowerSaturationLimit=-500
  Ki : Gain  Gain=1/rectifier.controller.VoltageT
  Kp : Gain  Gain=rectifier.controller.VoltageG
  Saturation : Saturate  UpperLimit=600  LowerLimit=-600
  Sum7 : Sum  Inputs=|++
  u : Outport  VectorParamsAs1DForOutWhenUnconnected=off
  wires:
  Integrator/1 -> Sum7/2
  Sum7/1 -> Saturation/1
  e/1 -> Kp/1
  Kp/1 -> Ki/1, Sum7/1
  Ki/1 -> Integrator/1
  Saturation/1 -> u/1

== system DCFastCharger/FEC control circuit/Controller/d-axis current control ==
  e : Inport
  Integrator : Integrator  LimitOutput=on  UpperSaturationLimit=10  LowerSaturationLimit=-10
  Ki : Gain  Gain=1/rectifier.controller.CurrentT
  Kp : Gain  Gain=rectifier.controller.CurrentG
  Saturation : Saturate  UpperLimit=4  LowerLimit=-4
  Sum7 : Sum  Inputs=|++
  u : Outport  VectorParamsAs1DForOutWhenUnconnected=off
  wires:
  Integrator/1 -> Sum7/2
  Sum7/1 -> Saturation/1
  e/1 -> Kp/1
  Kp/1 -> Ki/1, Sum7/1
  Ki/1 -> Integrator/1
  Saturation/1 -> u/1

== system DCFastCharger/FEC control circuit/Controller/q-axis current control ==
  e : Inport
  Integrator : Integrator  LimitOutput=on  UpperSaturationLimit=8  LowerSaturationLimit=-8
  Ki : Gain  Gain=1/rectifier.controller.CurrentT
  Kp : Gain  Gain=rectifier.controller.CurrentG
  Saturation : Saturate  UpperLimit=3  LowerLimit=-3
  Sum7 : Sum  Inputs=|++
  u : Outport  VectorParamsAs1DForOutWhenUnconnected=off
  wires:
  Ki/1 -> Integrator/1
  Kp/1 -> Sum7/1, Ki/1
  e/1 -> Kp/1
  Sum7/1 -> Saturation/1
  Saturation/1 -> u/1
  Integrator/1 -> Sum7/2

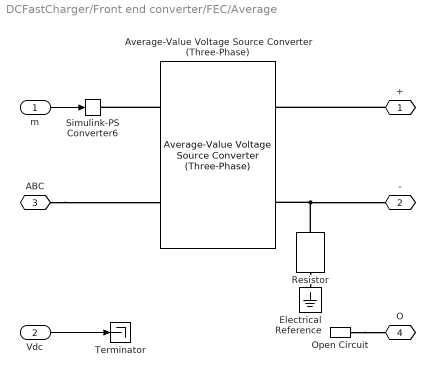
== system DCFastCharger/Front end converter/FEC/Average ==
  m : Inport
  Vdc : Inport  Port=2
  Average-Value Voltage Source Converter (Three-Phase) : ee_lib/Semiconductors & Converters/Converters/Average-Value Voltage Source Converter (Three-Phase)  port_option=ee.enum.threePhasePort.composite  enable_block_pulses_input=false  krec=0.01 Ohm  frequency_option=ee.enum.converters.frequency.variable  input_option=ee.enum.converters.inputOption.ModWave  FRated=60 Hz  losses_parameterization=ee.enum.converters.losses.fixed  Pfixed=1 W  ks=0.01  kc1=1.7 V  kc2=0.01 Ohm  Ploss_vect=[100, 800, 1870, 3250, 4900] W  Irms_vect=[10, 100, 200, 300, 400] A  Vdc_nom=300 V  thermal_mass=30000 J/K  temperature_specify=off  temperature_priority=High  temperature=298.15 K  temperature_nominal_specify=off  temperature_nominal_value=1  temperature_nominal_unit=K
  Electrical Reference : fl_lib/Electrical/Electrical Elements/Electrical Reference
  Open Circuit : fl_lib/Electrical/Electrical Elements/Open Circuit  v_specify=off  v_priority=None  v=0 V  v_nominal_specify=off  v_nominal_value=1  v_nominal_unit=V
  Resistor : fl_lib/Electrical/Electrical Elements/Resistor  R=1e6 Ohm  i_specify=off  i_priority=None  i=0 A  i_nominal_specify=off  i_nominal_value=1  i_nominal_unit=A  v_specify=off  v_priority=None  v=0 V  v_nominal_specify=off  v_nominal_value=1  v_nominal_unit=V
  Simulink-PS Converter6 : nesl_utility/Simulink-PS Converter  PhysicalDomain=network_engine_domain  SubClassName=ps_input  LeftPortType=input  RightPortType=output  PseudoPeriodic=off  Frequencies=[]  NoiseDistribution=none  NoiseParameters=[]  Unit=1  AffineConversion=off  FilteringAndDerivatives=provide  SimscapeFilterOrder=1  InputFilterTimeConstant=0.001  UdotUserProvided=0
  Terminator : Terminator
  + : PMIOPort  Side=Right
  - : PMIOPort  Port=2  Side=Right
  ABC : PMIOPort  Port=3  Side=Left
  O : PMIOPort  Port=4  Side=Right
  wires:
  m/1 -> Simulink-PS Converter6/1
  Vdc/1 -> Terminator/1
  connections:
  Open Circuit/LConn1 -- O/RConn1
  Average-Value Voltage Source Converter (Three-Phase)/LConn1 -- Simulink-PS Converter6/RConn1
  ABC/RConn1 -- Average-Value Voltage Source Converter (Three-Phase)/LConn2
  +/RConn1 -- Average-Value Voltage Source Converter (Three-Phase)/RConn1
  Resistor/LConn1 -- Average-Value Voltage Source Converter (Three-Phase)/RConn2 -- -/RConn1
  Resistor/RConn1 -- Electrical Reference/LConn1

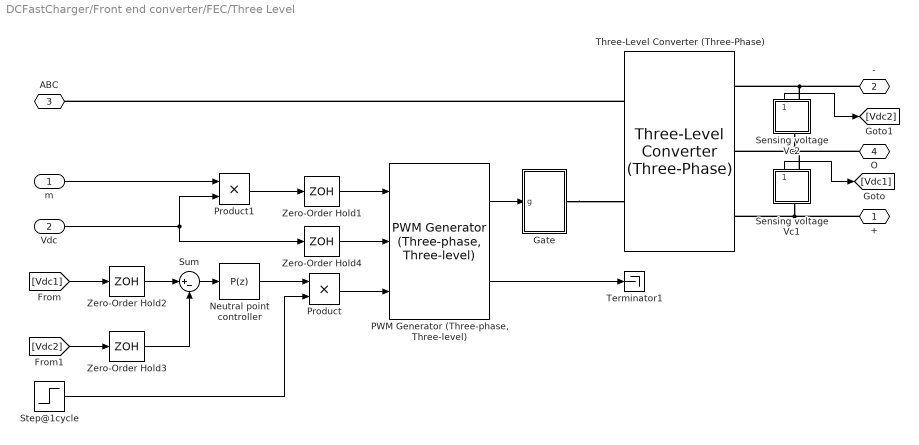
== system DCFastCharger/Front end converter/FEC/Three Level ==
  m : Inport
  Vdc : Inport  Port=2
  Gate : Subsystem
  Neutral point controller : slpidlib/PID Controller  Controller=P  Form=Parallel  TimeDomain=Discrete-time  UseExternalTs=off  SampleTime=-1  IntegratorMethod=Forward Euler  FilterMethod=Forward Euler  ControllerParametersSource=internal  P=0.001  I=80/2  UseKiTs=off  D=0  UseExternalDerivativeSource=off  N=100  UseFilter=on  TunerSelectOption=Transfer Function Based (PID Tuner App)  ZeroCross=off  InitialConditionSource=internal  InitialConditionForIntegrator=0  InitialConditionForFilter=0  DifferentiatorICPrevScaledInput=0  ExternalReset=none  TrackingMode=off  Kt=1  LimitOutput=on  SatLimitsSource=internal  UpperSaturationLimit=1  LowerSaturationLimit=-1  LinearizeAsGain=on  AntiWindupMode=back-calculation  Kb=1000  LimitIntegrator=off  UpperIntegratorSaturationLimit=inf  LowerIntegratorSaturationLimit=-inf  POutMin=[]  POutMax=[]  IOutMin=[]  IOutMax=[]  DOutMin=[]  DOutMax=[]  NOutMin=[]  NOutMax=[]  SumOutMin=[]  SumOutMax=[]  SaturationOutMin=[]  SaturationOutMax=[]  PParamMin=[]  PParamMax=[]  IParamMin=[]  IParamMax=[]  DParamMin=[]  DParamMax=[]  NParamMin=[]  NParamMax=[]  KbParamMin=[]  KbParamMax=[]  KtParamMin=[]  KtParamMax=[]  KbOutMin=[]  KbOutMax=[]  KtOutMin=[]  KtOutMax=[]  IntegratorOutMin=[]  IntegratorOutMax=[]  FilterOutMin=[]  FilterOutMax=[]  SumI1OutMin=[]  SumI1OutMax=[]  SumI2OutMin=[]  SumI2OutMax=[]  SumI3OutMin=[]  SumI3OutMax=[]  SumI4OutMin=[]  SumI4OutMax=[]  SumDOutMin=[]  SumDOutMax=[]  DifferentiatorOutMin=[]  DifferentiatorOutMax=[]  FilterDiffOutCoefMin=[]  FilterDiffOutCoefMax=[]  ReciprocalOutMin=[]  ReciprocalOutMax=[]  SumDenOutMin=[]  SumDenOutMax=[]  SumNumOutMin=[]  SumNumOutMax=[]  DivideOutMin=[]  DivideOutMax=[]  UdiffTsProdOutMin=[]  UdiffTsProdOutMax=[]  NTsProdOutMin=[]  NTsProdOutMax=[]  UintegralTsProdOutMin=[]  UintegralTsProdOutMax=[]  UngainTsProdOutMin=[]  UngainTsProdOutMax=[]  ClampingZeroOutDataTypeStr=Inherit: Inherit via back propagation  ClampingZeroOutMin=[]  ClampingZeroOutMax=[]  FilterDenConstantOutDataTypeStr=Inherit: Inherit via back propagation  FilterDenConstantOutMin=[]  FilterDenConstantOutMax=[]  PCopyOutDataTypeStr=Inherit: Inherit via back propagation  PCopyOutMin=[]  PCopyOutMax=[]  NCopyOutDataTypeStr=Inherit: Inherit via back propagation  NCopyOutMin=[]  NCopyOutMax=[]  IntegratorContinuousStateAttributes=''  IntegratorStateMustResolveToSignalObject=off  IntegratorRTWStateStorageClass=Auto  FilterContinuousStateAttributes=''  FilterStateMustResolveToSignalObject=off  FilterRTWStateStorageClass=Auto  ParallelPVariant=InternalParameters  IdealPVariant=Disabled  IVariant=Disabled  DVariant=Disabled  IntegratorVariant=Disabled  SatVariant=Enabled  AWVariant=Disabled  PCopyVariant=Disabled  TRVariant=Disabled  FdbkBlocksVariant=Forward  IdealPFdbkVariant=Disabled  SatFdbkVariant=Disabled  DerivativeFilterVariant=Disabled  NVariant=Disabled  NCopyVariant=Disabled_SignalSpec  FilterICVariant=Disabled  IntegratorICVariant=Disabled  ExternalResetVariant=Disabled  TRSumVariant=Passthrough  SumFdbkVariant=Disabled  SumVariant=Passthrough_P  TsampFilterVariant=InternalTs  TsampNgainVariant=Passthrough  TsampIntegralVariant=Disabled_SignalSpec  ExternalSaturationOutDataTypeStr=Inherit: Same as second input  DerivativeSourceVariant=Disabled  PreIntVariant=InternalPreInt
  "PWM Generator (Three-phase, Three-level)" : eePwmGeneratorThreeLevel/PWM Generator (Three-phase, Three-level)  CPWMMode=SPWM: sinusoidal PWM  fsw=rectifier.SwitchFrequency  Ts=1/(10*rectifier.SwitchFrequency)
      settings: SamplingMode=Natural
  Product : Product
  Product1 : Product
  Sensing voltage Vc1 : Subsystem
      mask Display: disp('Vdc1')
  Sensing voltage Vc2 : Subsystem
      mask Display: disp('Vdc2')
  Step@1cycle : Step  Time=1/rectifier.SystemFrequency  SampleTime=1/(10*rectifier.SwitchFrequency)
  Sum : Sum  Inputs=|+-
  Terminator1 : Terminator
  Three-Level Converter (Three-Phase) : ee_lib/Semiconductors & Converters/Converters/Three-Level Converter (Three-Phase)  port_option=ee.enum.threePhasePort.composite  device_type=2  Vf=0.8 V  Ron=0.001 Ohm  Rds=0.001 Ohm  Goff=1e-6 1/Ohm  Vth=0.2 V  Vgt=1 V  Vgt_off=-1 V  Ih=1 A  K=0  diode_param=2  diode_Vf=0.8 V  diode_Ron=0.001 Ohm  diode_Goff=1e-5 1/Ohm  diode_C=50 nF  diode_iRM=-235 A  diode_iF=300 A  diode_idot=-50 A/us  diode_trr_param=1  diode_trr_factor=3  diode_trr=15 us  diode_Qrr=1500 s*uA  snubber_type=0  Cs=1e-7 F  Rs=0.1 Ohm
  Zero-Order Hold1 : ZeroOrderHold  SampleTime=1/(10*rectifier.SwitchFrequency)
  Zero-Order Hold2 : ZeroOrderHold  SampleTime=1/(5*rectifier.SwitchFrequency)
  Zero-Order Hold3 : ZeroOrderHold  SampleTime=1/(5*rectifier.SwitchFrequency)
  Zero-Order Hold4 : ZeroOrderHold  SampleTime=1/(10*rectifier.SwitchFrequency)
  + : PMIOPort  Side=Right
  - : PMIOPort  Port=2  Side=Right
  ABC : PMIOPort  Port=3  Side=Left
  O : PMIOPort  Port=4  Side=Right
  wires:
  Sum/1 -> Neutral point controller/1
  Vdc/1 -> Zero-Order Hold4/1, Product1/2
  m/1 -> Product1/1
  Zero-Order Hold2/1 -> Sum/1
  Zero-Order Hold3/1 -> Sum/2
  Zero-Order Hold1/1 -> "PWM Generator (Three-phase, Three-level)"/1
  Zero-Order Hold4/1 -> "PWM Generator (Three-phase, Three-level)"/2
  "PWM Generator (Three-phase, Three-level)"/2 -> Terminator1/1
  Product1/1 -> Zero-Order Hold1/1
  [Vdc1] -> Zero-Order Hold2/1
  Step@1cycle/1 -> Product/2
  [Vdc2] -> Zero-Order Hold3/1
  Neutral point controller/1 -> Product/1
  Product/1 -> "PWM Generator (Three-phase, Three-level)"/3
  "PWM Generator (Three-phase, Three-level)"/1 -> Gate/1(g)
  Sensing voltage Vc1/1(Out1) -> [Vdc1]
  Sensing voltage Vc2/1(Out1) -> [Vdc2]
  connections:
  Sensing voltage Vc2/LConn1 -- Sensing voltage Vc1/RConn1 -- O/RConn1 -- Three-Level Converter (Three-Phase)/RConn2
  -/RConn1 -- Three-Level Converter (Three-Phase)/RConn3 -- Sensing voltage Vc2/RConn1
  +/RConn1 -- Three-Level Converter (Three-Phase)/RConn1 -- Sensing voltage Vc1/LConn1
  Three-Level Converter (Three-Phase)/LConn2 -- ABC/RConn1
  Gate/RConn1 -- Three-Level Converter (Three-Phase)/LConn1
